simulink model "simautoc1"  (Simulink 3.00)
settings: Solver=ode45  StartTime=0.0  StopTime=10  MaxStep=.01  RelTol=1e-6  AbsTol=1e-6
values from neighbouring files (symbols this model uses):
  Acon = [-2*k/(m*v), 0, 0, v/a-k/(m*v); v, 0, v, 0; 0, 0, 0, v/a; 0, 0, 0, 0]    [objauto2.m]
  Bcon = [0; 0; 0; 1]    [objauto2.m]
  Ccon = [0, 1, 0, 0]    [objauto2.m]
  Dcon = [0]    [objauto2.m]
  NoiseVariance = 0.001    [objauto2.m]
  STATEInit = [0, 1.0, 0, 0]    [objauto2.m]
  TIMEdis = 0.05    [objauto2.m]
undefined symbols (not defined in the file or in its folder): DenContr, NumContr
settings Model: SaveTime=off  SaveOutput=off  LastModifiedBy=pohlheim

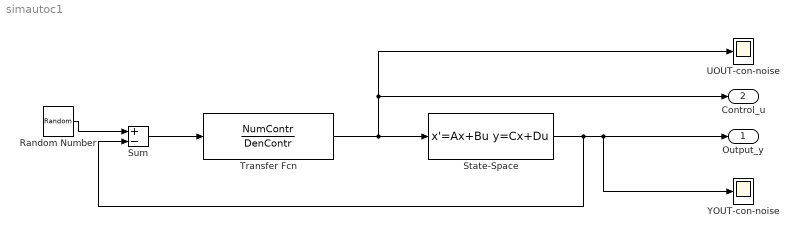
== system simautoc1 ==
  Random Number : RandomNumber  Mean=0  Variance=NoiseVariance  Seed=12345  SampleTime=TIMEdis
  State-Space : StateSpace  A=Acon  B=Bcon  C=Ccon  D=Dcon  X0=STATEInit
  Sum : Sum  Inputs=+-  SaturateOnIntegerOverflow=on
  Transfer Fcn : TransferFcn  Numerator=NumContr  Denominator=DenContr
  UOUT-con-noise : Scope
      settings: TimeRange=10  YMin=-0.1  YMax=0.1  SaveToWorkspace=off  SaveName=ScopeData  DataFormat=Matrix  LimitMaxRows=off  MaxRows=00
  YOUT-con-noise : Scope
      settings: TimeRange=11  YMin=-1  YMax=1  SaveToWorkspace=off  SaveName=ScopeData  DataFormat=Matrix  LimitMaxRows=off
  Output_y : Outport  Port=1
  Control_u : Outport  Port=2
  wires:
  Random Number/1 -> Sum/1
  Sum/1 -> Transfer Fcn/1
  Transfer Fcn/1 -> State-Space/1, Control_u/1, UOUT-con-noise/1
  State-Space/1 -> Output_y/1, YOUT-con-noise/1, Sum/2
